simulink model "practica2"  (R2026b)
settings: Solver=VariableStepAuto  StopTime=10
settings Model: Creator=diego  LastModifiedBy=diego

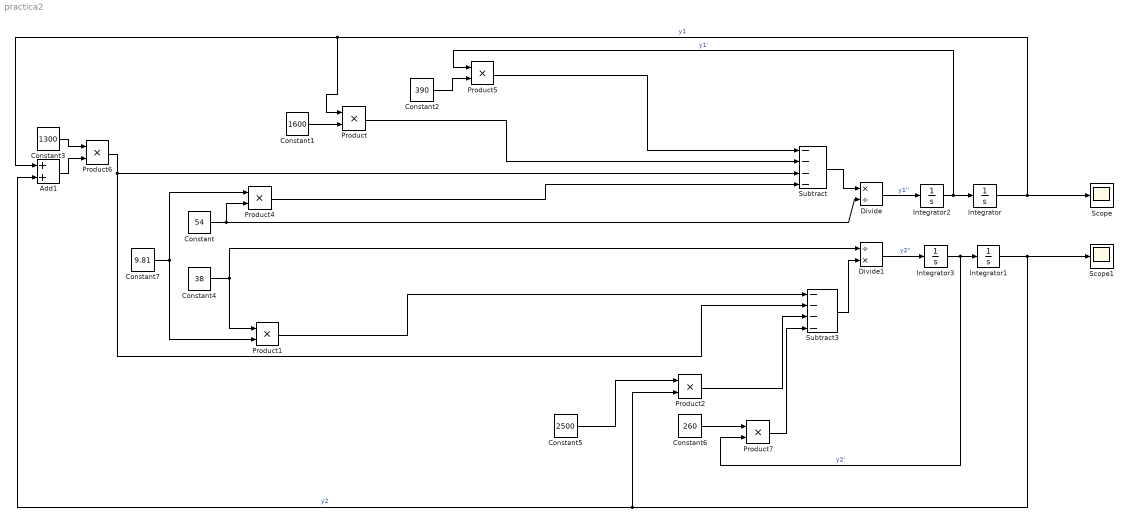
== system practica2 ==
  Add1 : Sum
  Constant : Constant  Value=54
  Constant1 : Constant  Value=1600
  Constant2 : Constant  Value=390
  Constant3 : Constant  Value=1300
  Constant4 : Constant  Value=38
  Constant5 : Constant  Value=2500
  Constant6 : Constant  Value=260
  Constant7 : Constant  Value=9.81
  Divide : Product  Inputs=*/
  Divide1 : Product  Inputs=/*
  Integrator{,1..3} (4 alike) : Integrator
  Product{,1..2,4..7} (7 alike) : Product
  Scope : Scope
      settings: ActiveDisplayYMinimum=-0.19474704291616682  ActiveDisplayYMaximum=0.021638560324018532
  Scope1 : Scope
      settings: ActiveDisplayYMinimum=-0.10629692674722913  ActiveDisplayYMaximum=0.01181076963858101
  Subtract : Sum  Inputs=----
  Subtract3 : Sum  Inputs=----
  wires:
  Integrator/1 -> Add1/1, Product/1, Scope/1  "y1"
  Integrator1/1 -> Product2/2, Add1/2, Scope1/1  "y2"
  Integrator2/1 -> Product5/1, Integrator/1  "y1'"
  Integrator3/1 -> Product7/2, Integrator1/1  "y2'"
  Divide/1 -> Integrator2/1  "y1''"
  Divide1/1 -> Integrator3/1  "y2''"
  Constant/1 -> Product4/2, Divide/2
  Constant4/1 -> Product1/1, Divide1/1
  Subtract/1 -> Divide/1
  Subtract3/1 -> Divide1/2
  Constant1/1 -> Product/2
  Product5/1 -> Subtract/1
  Constant7/1 -> Product1/2, Product4/1
  Product1/1 -> Subtract3/1
  Constant3/1 -> Product6/1
  Add1/1 -> Product6/2
  Product6/1 -> Subtract3/2, Subtract/3
  Product7/1 -> Subtract3/4
  Product2/1 -> Subtract3/3
  Constant5/1 -> Product2/1
  Constant6/1 -> Product7/1
  Product4/1 -> Subtract/4
  Constant2/1 -> Product5/2
  Product/1 -> Subtract/2
